simulink model "demoPassiveWavefilterAutopilot1"  (R2022a)
settings: Solver=ode4  StartTime=0.0  StopTime=1000  FixedStep=0.1  RelTol=1e-3  EnableMultiTasking=on
libraries: simulink_extras x5, mssSimulink x5, simulink x2
settings Model: Creator=Thor  LastModifiedBy=thor
settings SolverCC: AlgebraicLoopSolver=TrustRegion
settings DataIOCC: LimitDataPoints=on  SaveFormat=Array  SignalLoggingSaveFormat=ModelDataLogs  ReturnWorkspaceOutputs=off  SignalLoggingName=sigsOut
settings OptimizationCC: BooleanDataType=off  ExpressionDepthLimit=2147483647  InitFltsAndDblsToZero=on  LifeSpan=inf
settings DebuggingCC: SaveWithParameterizedLinksMsg=none  UnderspecifiedInitializationDetection=Classic  MergeDetectMultiDrivingBlocksExec=none  SignalResolutionControl=TryResolveAllWithWarning  MultiTaskDSMMsg=warning  MultiTaskCondExecSysMsg=none  FcnCallInpInsideContextMsg=warning  UnconnectedInputMsg=warning  UnconnectedOutputMsg=warning  UnconnectedLineMsg=warning  StateNameClashWarn=warning  SFUnexpectedBacktrackingDiag=warning  SFNoUnconditionalDefaultTransitionDiag=warning  SFExecutionAtInitializationDiag=none  SFMachineParentedDataDiag=warning  ArithmeticOperatorsInVariantConditions=warning
settings HardwareCC: ProdBitPerPointer=32  ProdBitPerSizeT=32  ProdBitPerPtrDiffT=32  ProdLargestAtomicFloat=None  ProdIntDivRoundTo=Undefined  ProdEndianess=Unspecified  ProdWordSize=32  ProdHWDeviceType=32-bit Generic  TargetUnknown=on
settings ModelReferenceCC: PropagateSignalLabelsOutOfModel=off
settings SFSimCC: SimUseLocalCustomCode=off  CustomCodeUndefinedFunction=UseInterfaceOnly
settings RTWCC: RTWUseLocalCustomCode=off  DLArmComputeVersion=19.05
settings CodeAppCC: StateflowObjectComments=on
settings GRTTargetCC: TargetFcnLib=ansi_tfl_tmw.mat  TargetLangStandard=C89/C90 (ANSI)  ModelReferenceCompliant=off  CombineOutputUpdateFcns=off  MatFileLogging=off  GRTInterface=on
settings ConfigComp: CovMetricSettings=dw  CovSaveCumulativeToWorkspaceVar=on  CovSaveSingleToWorkspaceVar=on  CovExternalEMLEnable=off

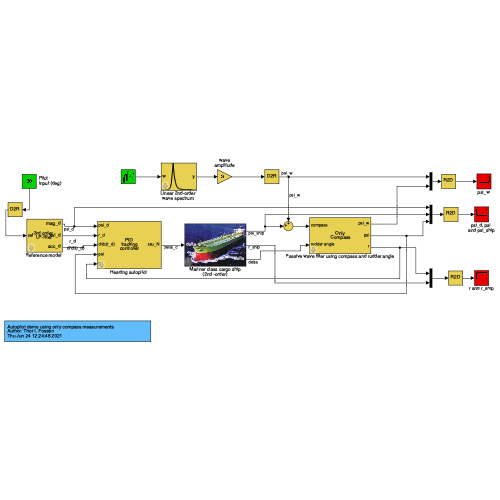
[thumbnail: Simulink's stored preview of the top-level diagram]
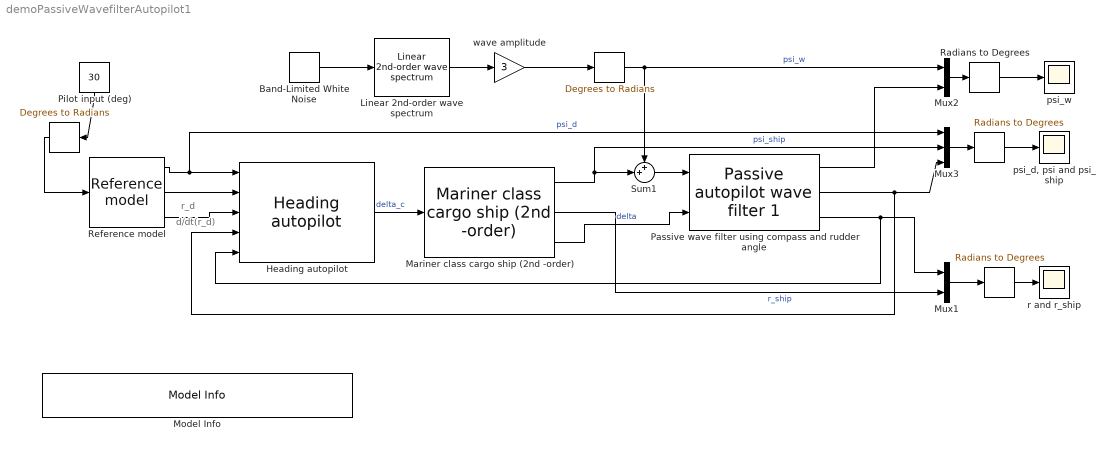
== system demoPassiveWavefilterAutopilot1 ==
  note: r_d
  note: d/dt(r_d)
  " " : simulink_extras/Transformations/Radians to Degrees
  "  " : simulink_extras/Transformations/Radians to Degrees
  "   " : simulink_extras/Transformations/Degrees to Radians
  "     " : simulink_extras/Transformations/Degrees to Radians
  Band-Limited White Noise : simulink/Sources/Band-Limited White Noise  Cov=[1]  Ts=0.1  seed=[23341]
  "Heading autopilot " : mssSimulink/Control/Autopilots/Heading autopilot  T_nomoto=107.3  K_nomoto=0.185  Kp=5  Td=10  Ti=100
  "Linear 2nd-order wave spectrum " : mssSimulink/Environment/Waves/Linear 2nd-order  wave spectrum  sigma=.5  w_0=1.2  lambda=0.1
  "Mariner class cargo ship (2nd -order) " : mssSimulink/Marine craft models/Mariner class cargo ship  (2nd -order)  rate_max=5*(pi/180)  delta_max=20*(pi/180)  K=0.185  T1=118  T2=7.8  T3=18.5
  Model Info : simulink/Model-Wide Utilities/Model Info  Frame=on  DisplayStringWithTags=|  HorizontalTextAlignment=Left  LeftAlignmentValue=0.02
      | Autopilot demo using only compass measurements
      | Author: Thor I. Fossen
      | %<LastModificationDate>
  Mux1 : Mux  Inputs=2
  Mux2 : Mux  Inputs=2
  Mux3 : Mux  Inputs=3
  Passive wave filter using compass and rudder angle : mssSimulink/Navigation/Estimators/Passive autopilot wave filter 1  lambda=0.1  w_o=1.2  K4=0.1  K5=0.01  w_c=1.3  T=107.3  K=0.185  T_b=100
  Pilot input (deg) : Constant  Value=30
  "Radians to Degrees  " : simulink_extras/Transformations/Radians to Degrees
  "Reference model " : mssSimulink/Guidance/Reference model  v_max=1.0  zeta_d=1.0  w_d=0.08
  Sum1 : Sum  Inputs=++|  InputSameDT=on  SaturateOnIntegerOverflow=on  OutDataTypeStr=Inherit: Same as first input
  "psi_d, psi and psi_ship" : Scope
  psi_w : Scope
  r and r_ship : Scope
  wave amplitude : Gain  Gain=3  SaturateOnIntegerOverflow=on  OutDataTypeStr=Inherit: Same as input  ParamDataTypeStr=Inherit: Same as input
  wires:
  Band-Limited White Noise/1 -> "Linear 2nd-order wave spectrum "/1
  Mux2/1 -> "Radians to Degrees  "/1
  "Radians to Degrees  "/1 -> psi_w/1
  " "/1 -> "psi_d, psi and psi_ship"/1
  Mux1/1 -> "  "/1
  "  "/1 -> r and r_ship/1
  "Linear 2nd-order wave spectrum "/1 -> wave amplitude/1
  Mux3/1 -> " "/1
  "Mariner class cargo ship (2nd -order) "/3 -> Passive wave filter using compass and rudder angle/2  "delta"
  wave amplitude/1 -> "   "/1
  "Heading autopilot "/1 -> "Mariner class cargo ship (2nd -order) "/1  "delta_c"
  Passive wave filter using compass and rudder angle/2 -> "Heading autopilot "/4, Mux3/3
  Passive wave filter using compass and rudder angle/3 -> "Heading autopilot "/5, Mux1/1
  "Mariner class cargo ship (2nd -order) "/1 -> Sum1/2, Mux3/2  "psi_ship"
  Sum1/1 -> Passive wave filter using compass and rudder angle/1
  "   "/1 -> Sum1/1, Mux2/1  "psi_w"
  "Mariner class cargo ship (2nd -order) "/2 -> Mux1/2  "r_ship"
  "Reference model "/1 -> "Heading autopilot "/1, Mux3/1  "psi_d"
  "Reference model "/2 -> "Heading autopilot "/2
  "Reference model "/3 -> "Heading autopilot "/3
  Passive wave filter using compass and rudder angle/1 -> Mux2/2
  Pilot input (deg)/1 -> "     "/1
  "     "/1 -> "Reference model "/1
